simulink model "plant_current_control"  (R2026b)
settings: Solver=VariableStepAuto  StopTime=100e-3
InitFcn:
  | parameters_current_control;
values from neighbouring files (symbols this model uses):
  A = -1/Tel    (= -250)    [parameters_current_control.m]
  B = 1/R*1/Tel    (= 166.666666667)    [parameters_current_control.m]
  C = 1    [parameters_current_control.m]
  D = 0    [parameters_current_control.m]
  L = 6e-3    (= 0.006)    [parameters_current_control.m]
  R = 1.5    [parameters_current_control.m]
  Tel = L/R    (= 0.004)    [parameters_current_control.m]
settings Model: Creator=ZAID  LastModifiedBy=ZAID

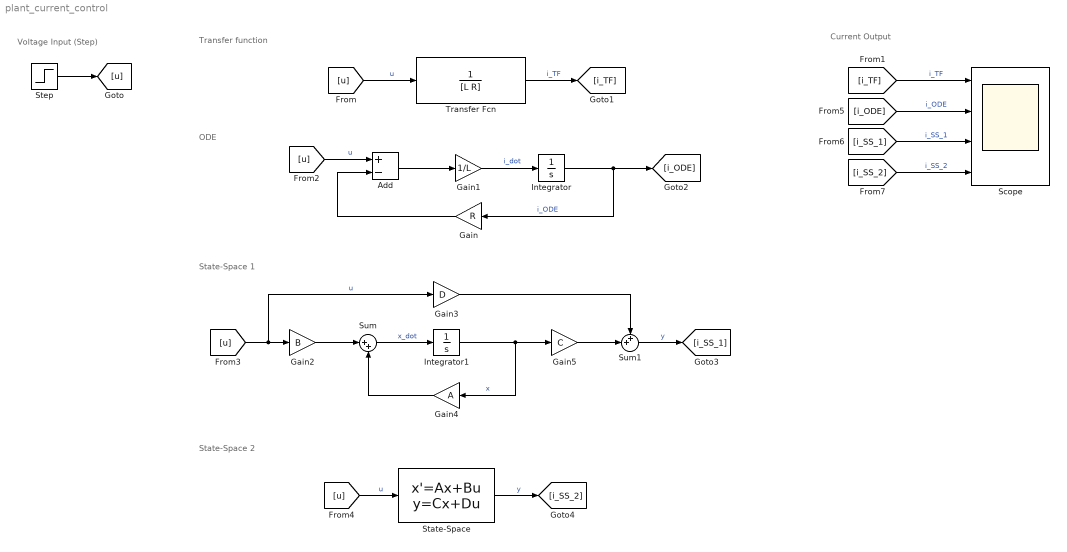
== system plant_current_control ==
  note: Current Output
  note: Voltage Input (Step)
  note: State-Space 2
  note: State-Space 1
  note: Transfer function
  note: ODE
  Add : Sum  Inputs=+-
  Gain : Gain  Gain=R
  Gain1 : Gain  Gain=1/L
  Gain2 : Gain  Gain=B
  Gain3 : Gain  Gain=D
  Gain4 : Gain  Gain=A
  Gain5 : Gain  Gain=C
  Integrator : Integrator
  Integrator1 : Integrator
  Scope : Scope  NumInputPorts=4
      settings: ActiveDisplayYMinimum=-0.083333333332175449  ActiveDisplayYMaximum=0.74999999998957922
  State-Space : StateSpace  A=-1/Tel  B=1/R*1/Tel  D=0  InitialCondition=0
  Step : Step  Time=0  SampleTime=0
  Sum : Sum  Inputs=|++
  Sum1 : Sum  Inputs=++|
  Transfer Fcn : TransferFcn  Denominator=[L R]
  wires:
  Integrator/1 -> [i_ODE], Gain/1  "i_ODE"
  Gain1/1 -> Integrator/1  "i_dot"
  Add/1 -> Gain1/1
  Gain/1 -> Add/2
  Integrator1/1 -> Gain4/1, Gain5/1  "x"
  Gain2/1 -> Sum/1
  Sum/1 -> Integrator1/1  "x_dot"
  Gain4/1 -> Sum/2
  Gain5/1 -> Sum1/2
  Gain3/1 -> Sum1/1
  Step/1 -> [u]
  [u] -> Transfer Fcn/1  "u"
  Transfer Fcn/1 -> [i_TF]  "i_TF"
  [i_TF] -> Scope/1  "i_TF"
  [u] -> Add/1  "u"
  [u] -> Gain2/1, Gain3/1  "u"
  Sum1/1 -> [i_SS_1]  "y"
  State-Space/1 -> [i_SS_2]  "y"
  [u] -> State-Space/1  "u"
  [i_ODE] -> Scope/2  "i_ODE"
  [i_SS_1] -> Scope/3  "i_SS_1"
  [i_SS_2] -> Scope/4  "i_SS_2"
